simulink subsystem "DualSpinTorque"  (R2024b)
settings: Solver=VariableStepAuto  StartTime=0.0  StopTime=10.0  RelTol=1e-3
settings Model: Creator=marco  LastModifiedBy=marco

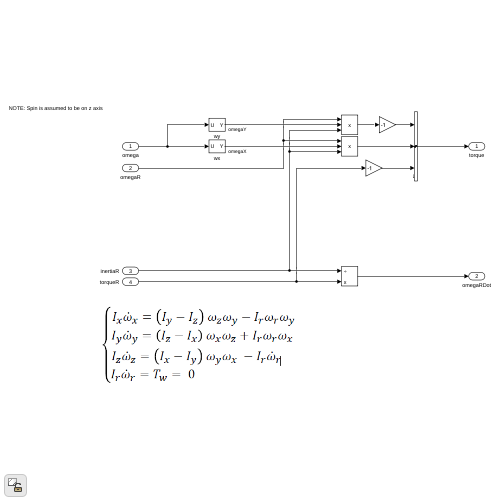
[thumbnail: Simulink's stored preview of the top-level diagram]
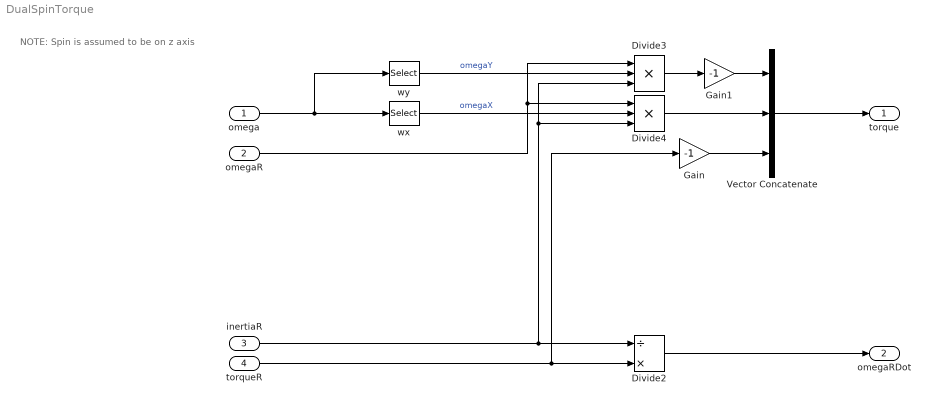
== system DualSpinTorque ==
  note: NOTE: Spin is assumed to be on z axis
  omega : Inport
  omegaR : Inport  Port=2
  inertiaR : Inport  Port=3
  torqueR : Inport  Port=4
  Divide2 : Product  Inputs=/*
  Divide3 : Product  Inputs=***
  Divide4 : Product  Inputs=***
  Gain : Gain  Gain=-1
  Gain1 : Gain  Gain=-1
  Vector Concatenate : Concatenate  NumInputs=3  Mode=Multidimensional array
  wx : Selector  NumberOfDimensions=2  InputPortWidth=3  IndexOptions=Index vector (dialog),Select all  Indices=1,1  OutputSizes=1,1
  wy : Selector  NumberOfDimensions=2  InputPortWidth=3  IndexOptions=Index vector (dialog),Select all  Indices=2,1  OutputSizes=1,1
  torque : Outport
  omegaRDot : Outport  Port=2
  wires:
  omega/1 -> wy/1, wx/1
  torqueR/1 -> Divide2/2, Gain/1
  inertiaR/1 -> Divide2/1, Divide4/3, Divide3/3
  omegaR/1 -> Divide4/1, Divide3/1
  wy/1 -> Divide3/2  "omegaY"
  wx/1 -> Divide4/2  "omegaX"
  Divide3/1 -> Gain1/1
  Divide4/1 -> Vector Concatenate/2
  Divide2/1 -> omegaRDot/1
  Vector Concatenate/1 -> torque/1
  Gain/1 -> Vector Concatenate/3
  Gain1/1 -> Vector Concatenate/1
